simulink model "exp3"  (R2018b)
settings: Solver=ode45  StartTime=0.0  StopTime=30  RelTol=1e-3
libraries: simulink x1
settings Model: Creator=lenovo  LastModifiedBy=lenovo

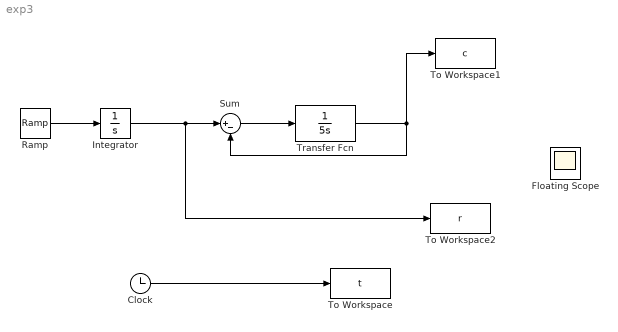
== system exp3 ==
  Clock : Clock
  Floating Scope : Scope
      settings: Floating=on
  Integrator : Integrator
  Ramp : simulink/Sources/Ramp  slope=1  start=0  InitialOutput=0
  Sum : Sum  Inputs=|+-
  To Workspace : ToWorkspace  VariableName=t  SampleTime=-1
  To Workspace1 : ToWorkspace  VariableName=c  SampleTime=-1
  To Workspace2 : ToWorkspace  VariableName=r  SampleTime=-1
  Transfer Fcn : TransferFcn  Denominator=[5 0]
  wires:
  Clock/1 -> To Workspace/1
  Transfer Fcn/1 -> To Workspace1/1, Sum/2
  Integrator/1 -> To Workspace2/1, Sum/1
  Sum/1 -> Transfer Fcn/1
  Ramp/1 -> Integrator/1
